simulink model "fw_closed_loop"  (R2024a)
settings: Solver=ode4  StartTime=0.0  StopTime=60  FixedStep=1e-3  RelTol=1e-3
settings Model: Creator=qixiaoyang  LastModifiedBy=qixiaoyang

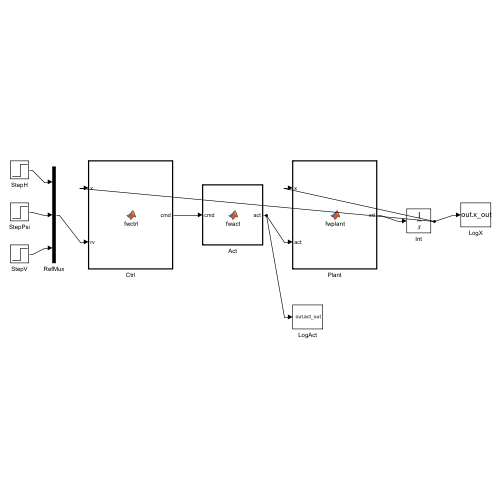
[thumbnail: Simulink's stored preview of the top-level diagram]
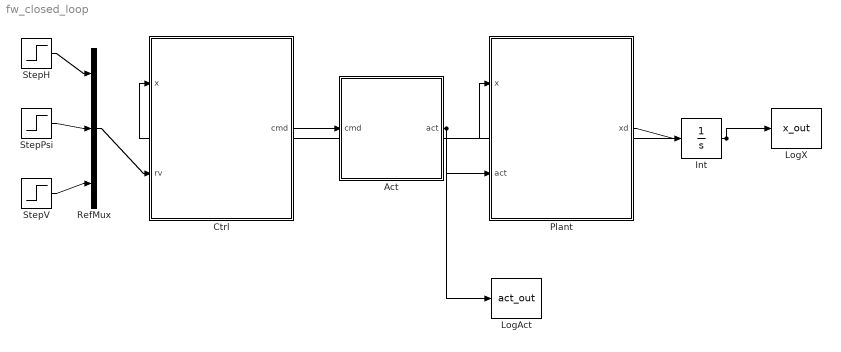
== system fw_closed_loop ==
  Act : MATLAB Function  TreatAsAtomicUnit=on
  Ctrl : MATLAB Function  TreatAsAtomicUnit=on
  Int : Integrator  InitialCondition=[0;0;-100;17.986780172076166;0;0.68973838620722472;0.99981637441965876;0;0.019162918418883054;0;0;0;0]
  LogAct : ToWorkspace  VariableName=act_out  SaveFormat=Timeseries  SampleTime=-1
  LogX : ToWorkspace  VariableName=x_out  SaveFormat=Timeseries  SampleTime=-1
  Plant : MATLAB Function  TreatAsAtomicUnit=on
  RefMux : Mux  Inputs=3
  StepH : Step  Time=5  Before=100  After=130  SampleTime=0
  StepPsi : Step  Time=20  After=1.0471975511965976  SampleTime=0
  StepV : Step  Time=35  Before=18  After=22  SampleTime=0
  wires:
  StepH/1 -> RefMux/1
  StepPsi/1 -> RefMux/2
  StepV/1 -> RefMux/3
  Int/1 -> Ctrl/1(x), Plant/1(x), LogX/1
  RefMux/1 -> Ctrl/2(rv)
  Ctrl/1(cmd) -> Act/1(cmd)
  Act/1(act) -> Plant/2(act), LogAct/1
  Plant/1(xd) -> Int/1

== matlab function fw_closed_loop/Ctrl ==
  settings: updateMethod=DISCRETE  sampleTime=1e-3
  data: x input; cmd output; rv input
function cmd = fwctrl(x, rv)
% 固定翼级联控制：高度-俯仰-升降舵、航向-滚转-副翼、速度-油门
persistent iV
if isempty(iV)
    iV = 0;
end
att = euler(x(7:10));
phi = att(1); theta = att(2); psi = att(3);
Vb = x(4:6);
V = max(norm(Vb), 1);
alpha = atan2(Vb(3), Vb(1));
p_ = x(11); q = x(12); r = x(13);
h = -x(3);
hdot = V*sin(theta - alpha);
ePsi = mod(rv(2) - psi + pi, 2*pi) - pi;
tr = trimV(rv(3));
aT = tr(1); deT = tr(2); thrT = tr(3);
eV = rv(3) - V;
iV = iV + 0.02*eV*0.001;
iV = min(max(iV, -0.29999999999999999), 0.29999999999999999);
thr = thrT + 0.14999999999999999*eV + iV;
thr = min(max(thr, 0), 1);
thCmd = aT + 0.029999999999999999*(rv(1) - h) - 0.040000000000000001*hdot;
thCmd = min(max(thCmd, -0.34999999999999998), 0.34999999999999998);
qCmd = 2*(thCmd - theta);
de = deT - 0.59999999999999998*(qCmd - q) - 0.5*(thCmd - theta);
phiCmd = 0.80000000000000004*ePsi;
phiCmd = min(max(phiCmd, -0.52000000000000002), 0.52000000000000002);
pCmd = 3*(phiCmd - phi);
da = 0.40000000000000002*(pCmd - p_);
dr = -0.5*r + 0.10000000000000001*phi;
cmd = [thr; min(max(de, -0.43633231299858238), 0.43633231299858238); min(max(da, -0.3490658503988659), 0.3490658503988659); min(max(dr, -0.43633231299858238), 0.43633231299858238)];
end
function tr = trimV(V)
% 定直平飞配平，返回 [alpha; de; thr]
qbar = 0.5*1.2250000000000001*V^2;
W = 5*9.8100000000000005;
CL = W/(qbar*0.55000000000000004);
for it = 1:6
    CD = 0.025000000000000001 + 0.044999999999999998*CL^2;
    D = qbar*0.55000000000000004*CD;
    A = [5 0.40000000000000002; -0.80000000000000004 -1.2];
    x = A \ [CL - 0.25; -0.050000000000000003];
    a = x(1);
    CL = (W*cos(a) - D*sin(a))/(qbar*0.55000000000000004*cos(a));
end
CD = 0.025000000000000001 + 0.044999999999999998*CL^2;
D = qbar*0.55000000000000004*CD;
L = qbar*0.55000000000000004*CL;
tr = [a; x(2); (D*cos(a) - L*sin(a) + W*sin(a))/40];
end
function e = euler(q)
n = norm(q);
if n < 1e-12, e = [0;0;0]; return; end
q = q/n;
w = q(1); x = q(2); y = q(3); z = q(4);
s2 = 2*(w*y - z*x);
s2 = max(-1, min(1, s2));
e = [atan2(2*(w*x + y*z), 1 - 2*(x*x + y*y));
     asin(s2);
     atan2(2*(w*z + x*y), 1 - 2*(y*y + z*z))];
end

== matlab function fw_closed_loop/Plant ==
  data: x input; xd output; act input
function xd = fwplant(x, act)
% 气动力/力矩 + 六自由度刚体方程
Vb = x(4:6); u = Vb(1); v = Vb(2); wb = Vb(3);
q = x(7:10); w = x(11:13);
m = 5;
g = 9.8100000000000005;
rho = 1.2250000000000001; S = 0.55000000000000004; b = 2.5; c = 0.22;
Tmax = 40;
thr = act(1); de = act(2); da = act(3); dr = act(4);
V = max(norm(Vb), 1);
alpha = asin(max(-0.34, min(0.34, wb/V)));
beta = asin(max(-0.34, min(0.34, v/V)));
qbar = 0.5*rho*V^2;
CL = 0.25 + 5*alpha + 3.8999999999999999*w(2)*c/(2*V) + 0.40000000000000002*de;
CD = 0.025000000000000001 + 0.044999999999999998*CL^2;
CY = -0.59999999999999998*beta + 0.19*dr;
Lft = qbar*S*CL; Dg = qbar*S*CD; Y = qbar*S*CY;
Xa = -Dg*cos(alpha) + Lft*sin(alpha);
Za = -Dg*sin(alpha) - Lft*cos(alpha);
Fb = [Xa + thr*Tmax; Y; Za];
Cl = -0.089999999999999997*beta + -0.5*w(1)*b/(2*V) + 0.080000000000000002*w(3)*b/(2*V) + 0.17999999999999999*da;
Cm = 0.050000000000000003 + -0.80000000000000004*alpha + -12*w(2)*c/(2*V) + -1.2*de;
Cn = 0.059999999999999998*beta + -0.029999999999999999*w(1)*b/(2*V) + -0.12*w(3)*b/(2*V) + 0.089999999999999997*dr;
Mb = [qbar*S*b*Cl; qbar*S*c*Cm; qbar*S*b*Cn];
R = dcm(q);
Vbd = Fb/m - cross(w, Vb) + R'*[0;0;g];
qd = 0.5*qmul(q, [0; w]);
I = [0.45000000000000001 0 0; 0 0.59999999999999998 0; 0 0 0.84999999999999998];
wd = I \ (Mb - cross(w, I*w));
xd = [R*Vb; Vbd; qd; wd];
end
function R = dcm(q)
n = norm(q);
if n < 1e-12, q = [1;0;0;0]; else, q = q/n; end
w = q(1); x = q(2); y = q(3); z = q(4);
R = [1-2*(y*y+z*z), 2*(x*y-w*z), 2*(x*z+w*y);
     2*(x*y+w*z), 1-2*(x*x+z*z), 2*(y*z-w*x);
     2*(x*z-w*y), 2*(y*z+w*x), 1-2*(x*x+y*y)];
end
function r = qmul(a, b)
aw = a(1); av = a(2:4);
bw = b(1); bv = b(2:4);
r = [aw*bw - av'*bv; aw*bv + bw*av + cross(av, bv)];
end

== matlab function fw_closed_loop/Act ==
  settings: updateMethod=DISCRETE  sampleTime=1e-3
  data: cmd input; act output
function act = fwact(cmd)
% 执行机构一阶滞后：每步更新一次，与 run_fw 的离散方式一致
persistent a
if isempty(a)
    a = [0.092939621189154262; 0.016114544747936877; 0; 0];
end
tau = [0.14999999999999999; 0.050000000000000003; 0.050000000000000003; 0.050000000000000003];
k = exp(-0.001 ./ tau);
a = cmd + (a - cmd).*k;
act = a;
end
